simulink library "casper_library_misc"  (Simulink 8.0)
settings: Solver=ode45  SolverMode=SingleTasking  StartTime=0.0  StopTime=10.0  RelTol=1e-3
libraries: xbsIndex_r4 x255, casper_library_misc x8, xps_library x6, simulink x4
(part 3 of 3)

== system casper_library_misc/complex_convert/ri_to_c ==
  re : Inport
  im : Inport  Port=2
  concat : xbsIndex_r4/Concat  num_inputs=2  dbl_ovrd=off  block_type=concat
      settings: block_version=9.1.01
  force_im : xbsIndex_r4/Reinterpret  force_arith_type=on  arith_type=Unsigned  force_bin_pt=on  bin_pt=0  block_type=reinterpret
      settings: infoedit="Changes signal type without altering the binary representation.   You can changed the signal between signed and unsigned, and relocate the binary point.<P><P>Hardware notes: In hardware this block costs nothing.<P><P>Example:  Suppose the input is 6 bits wide, signed, with 2 fractional bits, and the output is forced to unsigned with 0 fractional bits.  Then an input of -2.0 (1110.00 in binary 2's complement) becomes an output of 56 (111000 in binary)."  block_version=9.1.01
  force_re : xbsIndex_r4/Reinterpret  force_arith_type=on  arith_type=Unsigned  force_bin_pt=on  bin_pt=0  block_type=reinterpret
      settings: infoedit="Changes signal type without altering the binary representation.   You can changed the signal between signed and unsigned, and relocate the binary point.<P><P>Hardware notes: In hardware this block costs nothing.<P><P>Example:  Suppose the input is 6 bits wide, signed, with 2 fractional bits, and the output is forced to unsigned with 0 fractional bits.  Then an input of -2.0 (1110.00 in binary 2's complement) becomes an output of 56 (111000 in binary)."  block_version=9.1.01
  c : Outport
  wires:
  force_re/1 -> concat/1
  force_im/1 -> concat/2
  re/1 -> force_re/1
  concat/1 -> c/1
  im/1 -> force_im/1

== system casper_library_misc/pulse_ext/posedge ==
  In : Inport
  Delay : xbsIndex_r4/Delay  rst=off  infoeditControl=Selection of Reset will increase slice count due to use of real FFs and instead of SRLs  en=off  latency=1  dbl_ovrd=off  reg_retiming=on  block_type=delay
      settings: xl_area=[0, 0, 0, 0, 0, 0, 0]  block_version=9.1.01
  Inverter : xbsIndex_r4/Inverter  en=off  latency=0  dbl_ovrd=off  block_type=inv
      settings: xl_area=[0, 0, 0, 0, 0, 0, 0]  block_version=9.1.01
  Logical : xbsIndex_r4/Logical  logical_function=AND  inputs=2  en=off  latency=0  precision=Full  arith_type=Unsigned  n_bits=8  bin_pt=2  align_bp=on  dbl_ovrd=off  block_type=logical
      settings: xl_area=[0, 0, 0, 0, 0, 0, 0]  block_version=9.1.01
  Out : Outport
  wires:
  Logical/1 -> Out/1
  In/1 -> Logical/2, Delay/1
  Inverter/1 -> Logical/1
  Delay/1 -> Inverter/1

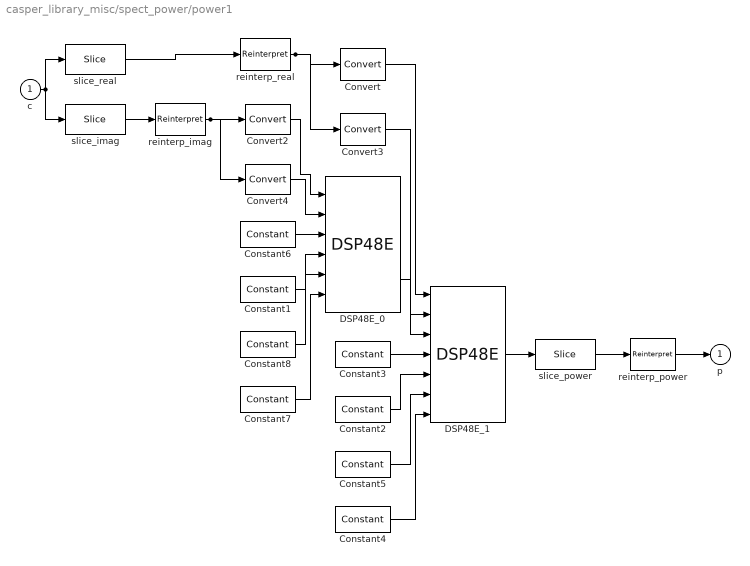
== system casper_library_misc/spect_power/power1 ==
  c : Inport
  Constant1 : xbsIndex_r4/Constant  const=0  gui_display_data_type=Fixed-point  arith_type=Unsigned  n_bits=4  bin_pt=0  preci_type=Single  exp_width=8  frac_width=24  explicit_period=off  period=1  equ=P=C  opselect=C  inp2=PCIN>>17  opr=+  inp1=P  carry=CIN  dbl_ovrd=off  block_type=constant
      settings: block_version=11.4
  Constant2 : xbsIndex_r4/Constant  const=0  gui_display_data_type=Fixed-point  arith_type=Unsigned  n_bits=4  bin_pt=0  preci_type=Single  exp_width=8  frac_width=24  explicit_period=off  period=1  equ=P=C  opselect=C  inp2=PCIN>>17  opr=+  inp1=P  carry=CIN  dbl_ovrd=off  block_type=constant
      settings: block_version=11.4
  Constant3 : xbsIndex_r4/Constant  const=21  gui_display_data_type=Fixed-point  arith_type=Unsigned  n_bits=7  bin_pt=0  preci_type=Single  exp_width=8  frac_width=24  explicit_period=off  period=1  equ=P=C  opselect=C  inp2=PCIN>>17  opr=+  inp1=P  carry=CIN  dbl_ovrd=off  block_type=constant
      settings: block_version=11.4
  Constant4 : xbsIndex_r4/Constant  const=0  gui_display_data_type=Fixed-point  arith_type=Unsigned  n_bits=3  bin_pt=0  preci_type=Single  exp_width=8  frac_width=24  explicit_period=off  period=1  equ=P=C  opselect=C  inp2=PCIN>>17  opr=+  inp1=P  carry=CIN  dbl_ovrd=off  block_type=constant
      settings: block_version=11.4
  Constant5 : xbsIndex_r4/Constant  const=0  gui_display_data_type=Fixed-point  arith_type=Unsigned  n_bits=1  bin_pt=0  preci_type=Single  exp_width=8  frac_width=24  explicit_period=off  period=1  equ=P=C  opselect=C  inp2=PCIN>>17  opr=+  inp1=P  carry=CIN  dbl_ovrd=off  block_type=constant
      settings: block_version=11.4
  Constant6 : xbsIndex_r4/Constant  const=5  gui_display_data_type=Fixed-point  arith_type=Unsigned  n_bits=7  bin_pt=0  preci_type=Single  exp_width=8  frac_width=24  explicit_period=off  period=1  equ=P=C  opselect=C  inp2=PCIN>>17  opr=+  inp1=P  carry=CIN  dbl_ovrd=off  block_type=constant
      settings: block_version=11.4
  Constant7 : xbsIndex_r4/Constant  const=0  gui_display_data_type=Fixed-point  arith_type=Unsigned  n_bits=3  bin_pt=0  preci_type=Single  exp_width=8  frac_width=24  explicit_period=off  period=1  equ=P=C  opselect=C  inp2=PCIN>>17  opr=+  inp1=P  carry=CIN  dbl_ovrd=off  block_type=constant
      settings: block_version=11.4
  Constant8 : xbsIndex_r4/Constant  const=0  gui_display_data_type=Fixed-point  arith_type=Unsigned  n_bits=1  bin_pt=0  preci_type=Single  exp_width=8  frac_width=24  explicit_period=off  period=1  equ=P=C  opselect=C  inp2=PCIN>>17  opr=+  inp1=P  carry=CIN  dbl_ovrd=off  block_type=constant
      settings: block_version=11.4
  Convert : xbsIndex_r4/Convert  gui_display_data_type=Fixed-point  arith_type="Signed  (2's comp)"  n_bits=30  bin_pt=0  float_type=Single  exp_bits=8  fraction_bits=24  quantization=Truncate  overflow=Wrap  en=off  latency=0  dbl_ovrd=off  pipeline=off  block_type=convert
      settings: block_version=11.4
  Convert2 : xbsIndex_r4/Convert  gui_display_data_type=Fixed-point  arith_type="Signed  (2's comp)"  n_bits=30  bin_pt=0  float_type=Single  exp_bits=8  fraction_bits=24  quantization=Truncate  overflow=Wrap  en=off  latency=0  dbl_ovrd=off  pipeline=off  block_type=convert
      settings: block_version=11.4
  Convert3 : xbsIndex_r4/Convert  gui_display_data_type=Fixed-point  arith_type="Signed  (2's comp)"  n_bits=18  bin_pt=0  float_type=Single  exp_bits=8  fraction_bits=24  quantization=Truncate  overflow=Wrap  en=off  latency=0  dbl_ovrd=off  pipeline=off  block_type=convert
      settings: block_version=11.4
  Convert4 : xbsIndex_r4/Convert  gui_display_data_type=Fixed-point  arith_type="Signed  (2's comp)"  n_bits=18  bin_pt=0  float_type=Single  exp_bits=8  fraction_bits=24  quantization=Truncate  overflow=Wrap  en=off  latency=0  dbl_ovrd=off  pipeline=off  block_type=convert
      settings: block_version=11.4
  DSP48E_0 : xbsIndex_r4/DSP48E  use_a=Direct from A Port  use_b=Direct from B Port  reset_preg=off  pattern_from_creg=off  pattern='000000000000'  mask_from_creg=off  pattern_mask='3FFFFFFFFFFF'  sel_rounding_mask=Select mask  use_op=off  use_creg=off  rst_all=off  en_all=off  use_pcin=off  use_carrycascin=off  use_multsignin=off  use_carryout=off  use_patterndetect=off  use_patternbdetect=off  use_overflow=off  use_underflow=off  use_acout=off  use_bcout=off  use_pcout=on  use_multsignout=off  use_carrycascout=off  pipeline_a=1  pipeline_b=1  pipeline_acout=1  pipeline_bcout=1  pipeline_c=on  pipeline_p=on  pipeline_mult=on  pipeline_opmode=on  pipeline_alumode=on  pipeline_carryin=on  pipeline_carryinsel=on  rst_a=off  rst_b=off  rst_c=off  rst_mult=off  rst_p=off  rst_carry_in=off  rst_alumode=off  rst_ctrl=off  en_a1=off  en_a2=off  en_b1=off  en_b2=off  en_c=off  en_mult=off  en_p=off  en_carry_in=off  en_alumode=off  en_multcarryin=off  en_ctrl=off  use_synth_model=off  addsub_mode=ONE48  xl_useadderonly=off  block_type=dsp48e
      settings: block_version=11.4
  DSP48E_1 : xbsIndex_r4/DSP48E  use_a=Direct from A Port  use_b=Direct from B Port  reset_preg=off  pattern_from_creg=off  pattern='000000000000'  mask_from_creg=off  pattern_mask='3FFFFFFFFFFF'  sel_rounding_mask=Select mask  use_op=off  use_creg=off  rst_all=off  en_all=off  use_pcin=on  use_carrycascin=off  use_multsignin=off  use_carryout=off  use_patterndetect=off  use_patternbdetect=off  use_overflow=off  use_underflow=off  use_acout=off  use_bcout=off  use_pcout=off  use_multsignout=off  use_carrycascout=off  pipeline_a=2  pipeline_b=2  pipeline_acout=1  pipeline_bcout=1  pipeline_c=on  pipeline_p=on  pipeline_mult=on  pipeline_opmode=on  pipeline_alumode=on  pipeline_carryin=on  pipeline_carryinsel=on  rst_a=off  rst_b=off  rst_c=off  rst_mult=off  rst_p=off  rst_carry_in=off  rst_alumode=off  rst_ctrl=off  en_a1=off  en_a2=off  en_b1=off  en_b2=off  en_c=off  en_mult=off  en_p=off  en_carry_in=off  en_alumode=off  en_multcarryin=off  en_ctrl=off  use_synth_model=off  addsub_mode=ONE48  xl_useadderonly=off  block_type=dsp48e
      settings: block_version=11.4
  reinterp_imag : xbsIndex_r4/Reinterpret  force_arith_type=on  arith_type="Signed  (2's comp)"  force_bin_pt=off  bin_pt=0  block_type=reinterpret
      settings: infoedit="Changes signal type without altering the binary representation.   You can changed the signal between signed and unsigned, and relocate the binary point.<br><br>Hardware notes: In hardware this block costs nothing.<br><br>Example:  Suppose the input is 6 bits wide, signed, with 2 fractional bits, and the output is forced to unsigned with 0 fractional bits.  Then an input of -2.0 (1110.00 in binary 2's complement) becomes an output of 56 (111000 in binary)."
  reinterp_power : xbsIndex_r4/Reinterpret  force_arith_type=on  arith_type=Unsigned  force_bin_pt=on  bin_pt=34  block_type=reinterpret
      settings: infoedit="Changes signal type without altering the binary representation.   You can changed the signal between signed and unsigned, and relocate the binary point.<br><br>Hardware notes: In hardware this block costs nothing.<br><br>Example:  Suppose the input is 6 bits wide, signed, with 2 fractional bits, and the output is forced to unsigned with 0 fractional bits.  Then an input of -2.0 (1110.00 in binary 2's complement) becomes an output of 56 (111000 in binary)."
  reinterp_real : xbsIndex_r4/Reinterpret  force_arith_type=on  arith_type="Signed  (2's comp)"  force_bin_pt=off  bin_pt=0  block_type=reinterpret
      settings: infoedit="Changes signal type without altering the binary representation.   You can changed the signal between signed and unsigned, and relocate the binary point.<br><br>Hardware notes: In hardware this block costs nothing.<br><br>Example:  Suppose the input is 6 bits wide, signed, with 2 fractional bits, and the output is forced to unsigned with 0 fractional bits.  Then an input of -2.0 (1110.00 in binary 2's complement) becomes an output of 56 (111000 in binary)."
  slice_imag : xbsIndex_r4/Slice  nbits=18  boolean_output=off  mode=Lower Bit Location + Width  bit1=0  base1=MSB of Input  bit0=0  base0=LSB of Input  dbl_ovrd=off  block_type=slice
  slice_power : xbsIndex_r4/Slice  nbits=36  boolean_output=off  mode=Lower Bit Location + Width  bit1=0  base1=MSB of Input  bit0=0  base0=LSB of Input  dbl_ovrd=off  block_type=slice
  slice_real : xbsIndex_r4/Slice  nbits=18  boolean_output=off  mode=Upper Bit Location + Width  bit1=0  base1=MSB of Input  bit0=0  base0=LSB of Input  dbl_ovrd=off  block_type=slice
  p : Outport
  wires:
  reinterp_imag/1 -> Convert4/1, Convert2/1
  reinterp_real/1 -> Convert3/1, Convert/1
  c/1 -> slice_real/1, slice_imag/1
  slice_real/1 -> reinterp_real/1
  slice_power/1 -> reinterp_power/1
  DSP48E_1/1 -> slice_power/1
  slice_imag/1 -> reinterp_imag/1
  reinterp_power/1 -> p/1
  Constant4/1 -> DSP48E_1/7
  Constant5/1 -> DSP48E_1/6
  Constant2/1 -> DSP48E_1/5
  Constant3/1 -> DSP48E_1/4
  DSP48E_0/2 -> DSP48E_1/3
  Convert3/1 -> DSP48E_1/2
  Convert/1 -> DSP48E_1/1
  Constant7/1 -> DSP48E_0/6
  Constant8/1 -> DSP48E_0/5
  Constant1/1 -> DSP48E_0/4
  Constant6/1 -> DSP48E_0/3
  Convert4/1 -> DSP48E_0/2
  Convert2/1 -> DSP48E_0/1

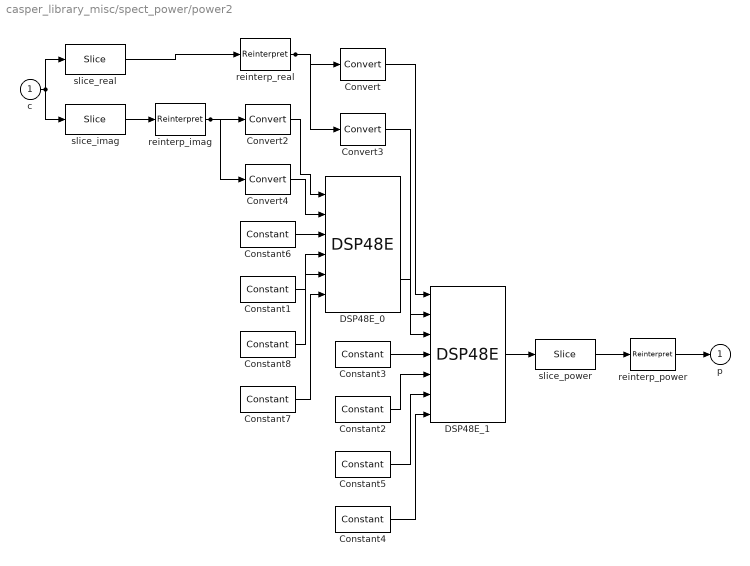
== system casper_library_misc/spect_power/power2 ==
  c : Inport
  Constant1 : xbsIndex_r4/Constant  const=0  gui_display_data_type=Fixed-point  arith_type=Unsigned  n_bits=4  bin_pt=0  preci_type=Single  exp_width=8  frac_width=24  explicit_period=off  period=1  equ=P=C  opselect=C  inp2=PCIN>>17  opr=+  inp1=P  carry=CIN  dbl_ovrd=off  block_type=constant
      settings: block_version=11.4
  Constant2 : xbsIndex_r4/Constant  const=0  gui_display_data_type=Fixed-point  arith_type=Unsigned  n_bits=4  bin_pt=0  preci_type=Single  exp_width=8  frac_width=24  explicit_period=off  period=1  equ=P=C  opselect=C  inp2=PCIN>>17  opr=+  inp1=P  carry=CIN  dbl_ovrd=off  block_type=constant
      settings: block_version=11.4
  Constant3 : xbsIndex_r4/Constant  const=21  gui_display_data_type=Fixed-point  arith_type=Unsigned  n_bits=7  bin_pt=0  preci_type=Single  exp_width=8  frac_width=24  explicit_period=off  period=1  equ=P=C  opselect=C  inp2=PCIN>>17  opr=+  inp1=P  carry=CIN  dbl_ovrd=off  block_type=constant
      settings: block_version=11.4
  Constant4 : xbsIndex_r4/Constant  const=0  gui_display_data_type=Fixed-point  arith_type=Unsigned  n_bits=3  bin_pt=0  preci_type=Single  exp_width=8  frac_width=24  explicit_period=off  period=1  equ=P=C  opselect=C  inp2=PCIN>>17  opr=+  inp1=P  carry=CIN  dbl_ovrd=off  block_type=constant
      settings: block_version=11.4
  Constant5 : xbsIndex_r4/Constant  const=0  gui_display_data_type=Fixed-point  arith_type=Unsigned  n_bits=1  bin_pt=0  preci_type=Single  exp_width=8  frac_width=24  explicit_period=off  period=1  equ=P=C  opselect=C  inp2=PCIN>>17  opr=+  inp1=P  carry=CIN  dbl_ovrd=off  block_type=constant
      settings: block_version=11.4
  Constant6 : xbsIndex_r4/Constant  const=5  gui_display_data_type=Fixed-point  arith_type=Unsigned  n_bits=7  bin_pt=0  preci_type=Single  exp_width=8  frac_width=24  explicit_period=off  period=1  equ=P=C  opselect=C  inp2=PCIN>>17  opr=+  inp1=P  carry=CIN  dbl_ovrd=off  block_type=constant
      settings: block_version=11.4
  Constant7 : xbsIndex_r4/Constant  const=0  gui_display_data_type=Fixed-point  arith_type=Unsigned  n_bits=3  bin_pt=0  preci_type=Single  exp_width=8  frac_width=24  explicit_period=off  period=1  equ=P=C  opselect=C  inp2=PCIN>>17  opr=+  inp1=P  carry=CIN  dbl_ovrd=off  block_type=constant
      settings: block_version=11.4
  Constant8 : xbsIndex_r4/Constant  const=0  gui_display_data_type=Fixed-point  arith_type=Unsigned  n_bits=1  bin_pt=0  preci_type=Single  exp_width=8  frac_width=24  explicit_period=off  period=1  equ=P=C  opselect=C  inp2=PCIN>>17  opr=+  inp1=P  carry=CIN  dbl_ovrd=off  block_type=constant
      settings: block_version=11.4
  Convert : xbsIndex_r4/Convert  gui_display_data_type=Fixed-point  arith_type="Signed  (2's comp)"  n_bits=30  bin_pt=0  float_type=Single  exp_bits=8  fraction_bits=24  quantization=Truncate  overflow=Wrap  en=off  latency=0  dbl_ovrd=off  pipeline=off  block_type=convert
      settings: block_version=11.4
  Convert2 : xbsIndex_r4/Convert  gui_display_data_type=Fixed-point  arith_type="Signed  (2's comp)"  n_bits=30  bin_pt=0  float_type=Single  exp_bits=8  fraction_bits=24  quantization=Truncate  overflow=Wrap  en=off  latency=0  dbl_ovrd=off  pipeline=off  block_type=convert
      settings: block_version=11.4
  Convert3 : xbsIndex_r4/Convert  gui_display_data_type=Fixed-point  arith_type="Signed  (2's comp)"  n_bits=18  bin_pt=0  float_type=Single  exp_bits=8  fraction_bits=24  quantization=Truncate  overflow=Wrap  en=off  latency=0  dbl_ovrd=off  pipeline=off  block_type=convert
      settings: block_version=11.4
  Convert4 : xbsIndex_r4/Convert  gui_display_data_type=Fixed-point  arith_type="Signed  (2's comp)"  n_bits=18  bin_pt=0  float_type=Single  exp_bits=8  fraction_bits=24  quantization=Truncate  overflow=Wrap  en=off  latency=0  dbl_ovrd=off  pipeline=off  block_type=convert
      settings: block_version=11.4
  DSP48E_0 : xbsIndex_r4/DSP48E  use_a=Direct from A Port  use_b=Direct from B Port  reset_preg=off  pattern_from_creg=off  pattern='000000000000'  mask_from_creg=off  pattern_mask='3FFFFFFFFFFF'  sel_rounding_mask=Select mask  use_op=off  use_creg=off  rst_all=off  en_all=off  use_pcin=off  use_carrycascin=off  use_multsignin=off  use_carryout=off  use_patterndetect=off  use_patternbdetect=off  use_overflow=off  use_underflow=off  use_acout=off  use_bcout=off  use_pcout=on  use_multsignout=off  use_carrycascout=off  pipeline_a=1  pipeline_b=1  pipeline_acout=1  pipeline_bcout=1  pipeline_c=on  pipeline_p=on  pipeline_mult=on  pipeline_opmode=on  pipeline_alumode=on  pipeline_carryin=on  pipeline_carryinsel=on  rst_a=off  rst_b=off  rst_c=off  rst_mult=off  rst_p=off  rst_carry_in=off  rst_alumode=off  rst_ctrl=off  en_a1=off  en_a2=off  en_b1=off  en_b2=off  en_c=off  en_mult=off  en_p=off  en_carry_in=off  en_alumode=off  en_multcarryin=off  en_ctrl=off  use_synth_model=off  addsub_mode=ONE48  xl_useadderonly=off  block_type=dsp48e
      settings: block_version=11.4
  DSP48E_1 : xbsIndex_r4/DSP48E  use_a=Direct from A Port  use_b=Direct from B Port  reset_preg=off  pattern_from_creg=off  pattern='000000000000'  mask_from_creg=off  pattern_mask='3FFFFFFFFFFF'  sel_rounding_mask=Select mask  use_op=off  use_creg=off  rst_all=off  en_all=off  use_pcin=on  use_carrycascin=off  use_multsignin=off  use_carryout=off  use_patterndetect=off  use_patternbdetect=off  use_overflow=off  use_underflow=off  use_acout=off  use_bcout=off  use_pcout=off  use_multsignout=off  use_carrycascout=off  pipeline_a=2  pipeline_b=2  pipeline_acout=1  pipeline_bcout=1  pipeline_c=on  pipeline_p=on  pipeline_mult=on  pipeline_opmode=on  pipeline_alumode=on  pipeline_carryin=on  pipeline_carryinsel=on  rst_a=off  rst_b=off  rst_c=off  rst_mult=off  rst_p=off  rst_carry_in=off  rst_alumode=off  rst_ctrl=off  en_a1=off  en_a2=off  en_b1=off  en_b2=off  en_c=off  en_mult=off  en_p=off  en_carry_in=off  en_alumode=off  en_multcarryin=off  en_ctrl=off  use_synth_model=off  addsub_mode=ONE48  xl_useadderonly=off  block_type=dsp48e
      settings: block_version=11.4
  reinterp_imag : xbsIndex_r4/Reinterpret  force_arith_type=on  arith_type="Signed  (2's comp)"  force_bin_pt=off  bin_pt=0  block_type=reinterpret
      settings: infoedit="Changes signal type without altering the binary representation.   You can changed the signal between signed and unsigned, and relocate the binary point.<br><br>Hardware notes: In hardware this block costs nothing.<br><br>Example:  Suppose the input is 6 bits wide, signed, with 2 fractional bits, and the output is forced to unsigned with 0 fractional bits.  Then an input of -2.0 (1110.00 in binary 2's complement) becomes an output of 56 (111000 in binary)."
  reinterp_power : xbsIndex_r4/Reinterpret  force_arith_type=on  arith_type=Unsigned  force_bin_pt=on  bin_pt=34  block_type=reinterpret
      settings: infoedit="Changes signal type without altering the binary representation.   You can changed the signal between signed and unsigned, and relocate the binary point.<br><br>Hardware notes: In hardware this block costs nothing.<br><br>Example:  Suppose the input is 6 bits wide, signed, with 2 fractional bits, and the output is forced to unsigned with 0 fractional bits.  Then an input of -2.0 (1110.00 in binary 2's complement) becomes an output of 56 (111000 in binary)."
  reinterp_real : xbsIndex_r4/Reinterpret  force_arith_type=on  arith_type="Signed  (2's comp)"  force_bin_pt=off  bin_pt=0  block_type=reinterpret
      settings: infoedit="Changes signal type without altering the binary representation.   You can changed the signal between signed and unsigned, and relocate the binary point.<br><br>Hardware notes: In hardware this block costs nothing.<br><br>Example:  Suppose the input is 6 bits wide, signed, with 2 fractional bits, and the output is forced to unsigned with 0 fractional bits.  Then an input of -2.0 (1110.00 in binary 2's complement) becomes an output of 56 (111000 in binary)."
  slice_imag : xbsIndex_r4/Slice  nbits=18  boolean_output=off  mode=Lower Bit Location + Width  bit1=0  base1=MSB of Input  bit0=0  base0=LSB of Input  dbl_ovrd=off  block_type=slice
  slice_power : xbsIndex_r4/Slice  nbits=36  boolean_output=off  mode=Lower Bit Location + Width  bit1=0  base1=MSB of Input  bit0=0  base0=LSB of Input  dbl_ovrd=off  block_type=slice
  slice_real : xbsIndex_r4/Slice  nbits=18  boolean_output=off  mode=Upper Bit Location + Width  bit1=0  base1=MSB of Input  bit0=0  base0=LSB of Input  dbl_ovrd=off  block_type=slice
  p : Outport
  wires:
  reinterp_imag/1 -> Convert4/1, Convert2/1
  reinterp_real/1 -> Convert3/1, Convert/1
  c/1 -> slice_real/1, slice_imag/1
  slice_real/1 -> reinterp_real/1
  slice_power/1 -> reinterp_power/1
  DSP48E_1/1 -> slice_power/1
  slice_imag/1 -> reinterp_imag/1
  reinterp_power/1 -> p/1
  Constant4/1 -> DSP48E_1/7
  Constant5/1 -> DSP48E_1/6
  Constant2/1 -> DSP48E_1/5
  Constant3/1 -> DSP48E_1/4
  DSP48E_0/2 -> DSP48E_1/3
  Convert3/1 -> DSP48E_1/2
  Convert/1 -> DSP48E_1/1
  Constant7/1 -> DSP48E_0/6
  Constant8/1 -> DSP48E_0/5
  Constant1/1 -> DSP48E_0/4
  Constant6/1 -> DSP48E_0/3
  Convert4/1 -> DSP48E_0/2
  Convert2/1 -> DSP48E_0/1

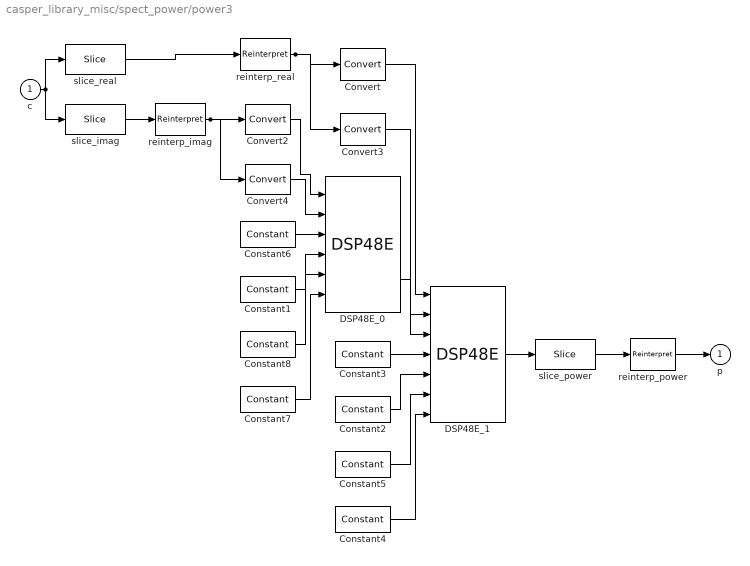
== system casper_library_misc/spect_power/power3 ==
  c : Inport
  Constant1 : xbsIndex_r4/Constant  const=0  gui_display_data_type=Fixed-point  arith_type=Unsigned  n_bits=4  bin_pt=0  preci_type=Single  exp_width=8  frac_width=24  explicit_period=off  period=1  equ=P=C  opselect=C  inp2=PCIN>>17  opr=+  inp1=P  carry=CIN  dbl_ovrd=off  block_type=constant
      settings: block_version=11.4
  Constant2 : xbsIndex_r4/Constant  const=0  gui_display_data_type=Fixed-point  arith_type=Unsigned  n_bits=4  bin_pt=0  preci_type=Single  exp_width=8  frac_width=24  explicit_period=off  period=1  equ=P=C  opselect=C  inp2=PCIN>>17  opr=+  inp1=P  carry=CIN  dbl_ovrd=off  block_type=constant
      settings: block_version=11.4
  Constant3 : xbsIndex_r4/Constant  const=21  gui_display_data_type=Fixed-point  arith_type=Unsigned  n_bits=7  bin_pt=0  preci_type=Single  exp_width=8  frac_width=24  explicit_period=off  period=1  equ=P=C  opselect=C  inp2=PCIN>>17  opr=+  inp1=P  carry=CIN  dbl_ovrd=off  block_type=constant
      settings: block_version=11.4
  Constant4 : xbsIndex_r4/Constant  const=0  gui_display_data_type=Fixed-point  arith_type=Unsigned  n_bits=3  bin_pt=0  preci_type=Single  exp_width=8  frac_width=24  explicit_period=off  period=1  equ=P=C  opselect=C  inp2=PCIN>>17  opr=+  inp1=P  carry=CIN  dbl_ovrd=off  block_type=constant
      settings: block_version=11.4
  Constant5 : xbsIndex_r4/Constant  const=0  gui_display_data_type=Fixed-point  arith_type=Unsigned  n_bits=1  bin_pt=0  preci_type=Single  exp_width=8  frac_width=24  explicit_period=off  period=1  equ=P=C  opselect=C  inp2=PCIN>>17  opr=+  inp1=P  carry=CIN  dbl_ovrd=off  block_type=constant
      settings: block_version=11.4
  Constant6 : xbsIndex_r4/Constant  const=5  gui_display_data_type=Fixed-point  arith_type=Unsigned  n_bits=7  bin_pt=0  preci_type=Single  exp_width=8  frac_width=24  explicit_period=off  period=1  equ=P=C  opselect=C  inp2=PCIN>>17  opr=+  inp1=P  carry=CIN  dbl_ovrd=off  block_type=constant
      settings: block_version=11.4
  Constant7 : xbsIndex_r4/Constant  const=0  gui_display_data_type=Fixed-point  arith_type=Unsigned  n_bits=3  bin_pt=0  preci_type=Single  exp_width=8  frac_width=24  explicit_period=off  period=1  equ=P=C  opselect=C  inp2=PCIN>>17  opr=+  inp1=P  carry=CIN  dbl_ovrd=off  block_type=constant
      settings: block_version=11.4
  Constant8 : xbsIndex_r4/Constant  const=0  gui_display_data_type=Fixed-point  arith_type=Unsigned  n_bits=1  bin_pt=0  preci_type=Single  exp_width=8  frac_width=24  explicit_period=off  period=1  equ=P=C  opselect=C  inp2=PCIN>>17  opr=+  inp1=P  carry=CIN  dbl_ovrd=off  block_type=constant
      settings: block_version=11.4
  Convert : xbsIndex_r4/Convert  gui_display_data_type=Fixed-point  arith_type="Signed  (2's comp)"  n_bits=30  bin_pt=0  float_type=Single  exp_bits=8  fraction_bits=24  quantization=Truncate  overflow=Wrap  en=off  latency=0  dbl_ovrd=off  pipeline=off  block_type=convert
      settings: block_version=11.4
  Convert2 : xbsIndex_r4/Convert  gui_display_data_type=Fixed-point  arith_type="Signed  (2's comp)"  n_bits=30  bin_pt=0  float_type=Single  exp_bits=8  fraction_bits=24  quantization=Truncate  overflow=Wrap  en=off  latency=0  dbl_ovrd=off  pipeline=off  block_type=convert
      settings: block_version=11.4
  Convert3 : xbsIndex_r4/Convert  gui_display_data_type=Fixed-point  arith_type="Signed  (2's comp)"  n_bits=18  bin_pt=0  float_type=Single  exp_bits=8  fraction_bits=24  quantization=Truncate  overflow=Wrap  en=off  latency=0  dbl_ovrd=off  pipeline=off  block_type=convert
      settings: block_version=11.4
  Convert4 : xbsIndex_r4/Convert  gui_display_data_type=Fixed-point  arith_type="Signed  (2's comp)"  n_bits=18  bin_pt=0  float_type=Single  exp_bits=8  fraction_bits=24  quantization=Truncate  overflow=Wrap  en=off  latency=0  dbl_ovrd=off  pipeline=off  block_type=convert
      settings: block_version=11.4
  DSP48E_0 : xbsIndex_r4/DSP48E  use_a=Direct from A Port  use_b=Direct from B Port  reset_preg=off  pattern_from_creg=off  pattern='000000000000'  mask_from_creg=off  pattern_mask='3FFFFFFFFFFF'  sel_rounding_mask=Select mask  use_op=off  use_creg=off  rst_all=off  en_all=off  use_pcin=off  use_carrycascin=off  use_multsignin=off  use_carryout=off  use_patterndetect=off  use_patternbdetect=off  use_overflow=off  use_underflow=off  use_acout=off  use_bcout=off  use_pcout=on  use_multsignout=off  use_carrycascout=off  pipeline_a=1  pipeline_b=1  pipeline_acout=1  pipeline_bcout=1  pipeline_c=on  pipeline_p=on  pipeline_mult=on  pipeline_opmode=on  pipeline_alumode=on  pipeline_carryin=on  pipeline_carryinsel=on  rst_a=off  rst_b=off  rst_c=off  rst_mult=off  rst_p=off  rst_carry_in=off  rst_alumode=off  rst_ctrl=off  en_a1=off  en_a2=off  en_b1=off  en_b2=off  en_c=off  en_mult=off  en_p=off  en_carry_in=off  en_alumode=off  en_multcarryin=off  en_ctrl=off  use_synth_model=off  addsub_mode=ONE48  xl_useadderonly=off  block_type=dsp48e
      settings: block_version=11.4
  DSP48E_1 : xbsIndex_r4/DSP48E  use_a=Direct from A Port  use_b=Direct from B Port  reset_preg=off  pattern_from_creg=off  pattern='000000000000'  mask_from_creg=off  pattern_mask='3FFFFFFFFFFF'  sel_rounding_mask=Select mask  use_op=off  use_creg=off  rst_all=off  en_all=off  use_pcin=on  use_carrycascin=off  use_multsignin=off  use_carryout=off  use_patterndetect=off  use_patternbdetect=off  use_overflow=off  use_underflow=off  use_acout=off  use_bcout=off  use_pcout=off  use_multsignout=off  use_carrycascout=off  pipeline_a=2  pipeline_b=2  pipeline_acout=1  pipeline_bcout=1  pipeline_c=on  pipeline_p=on  pipeline_mult=on  pipeline_opmode=on  pipeline_alumode=on  pipeline_carryin=on  pipeline_carryinsel=on  rst_a=off  rst_b=off  rst_c=off  rst_mult=off  rst_p=off  rst_carry_in=off  rst_alumode=off  rst_ctrl=off  en_a1=off  en_a2=off  en_b1=off  en_b2=off  en_c=off  en_mult=off  en_p=off  en_carry_in=off  en_alumode=off  en_multcarryin=off  en_ctrl=off  use_synth_model=off  addsub_mode=ONE48  xl_useadderonly=off  block_type=dsp48e
      settings: block_version=11.4
  reinterp_imag : xbsIndex_r4/Reinterpret  force_arith_type=on  arith_type="Signed  (2's comp)"  force_bin_pt=off  bin_pt=0  block_type=reinterpret
      settings: infoedit="Changes signal type without altering the binary representation.   You can changed the signal between signed and unsigned, and relocate the binary point.<br><br>Hardware notes: In hardware this block costs nothing.<br><br>Example:  Suppose the input is 6 bits wide, signed, with 2 fractional bits, and the output is forced to unsigned with 0 fractional bits.  Then an input of -2.0 (1110.00 in binary 2's complement) becomes an output of 56 (111000 in binary)."
  reinterp_power : xbsIndex_r4/Reinterpret  force_arith_type=on  arith_type=Unsigned  force_bin_pt=on  bin_pt=34  block_type=reinterpret
      settings: infoedit="Changes signal type without altering the binary representation.   You can changed the signal between signed and unsigned, and relocate the binary point.<br><br>Hardware notes: In hardware this block costs nothing.<br><br>Example:  Suppose the input is 6 bits wide, signed, with 2 fractional bits, and the output is forced to unsigned with 0 fractional bits.  Then an input of -2.0 (1110.00 in binary 2's complement) becomes an output of 56 (111000 in binary)."
  reinterp_real : xbsIndex_r4/Reinterpret  force_arith_type=on  arith_type="Signed  (2's comp)"  force_bin_pt=off  bin_pt=0  block_type=reinterpret
      settings: infoedit="Changes signal type without altering the binary representation.   You can changed the signal between signed and unsigned, and relocate the binary point.<br><br>Hardware notes: In hardware this block costs nothing.<br><br>Example:  Suppose the input is 6 bits wide, signed, with 2 fractional bits, and the output is forced to unsigned with 0 fractional bits.  Then an input of -2.0 (1110.00 in binary 2's complement) becomes an output of 56 (111000 in binary)."
  slice_imag : xbsIndex_r4/Slice  nbits=18  boolean_output=off  mode=Lower Bit Location + Width  bit1=0  base1=MSB of Input  bit0=0  base0=LSB of Input  dbl_ovrd=off  block_type=slice
  slice_power : xbsIndex_r4/Slice  nbits=36  boolean_output=off  mode=Lower Bit Location + Width  bit1=0  base1=MSB of Input  bit0=0  base0=LSB of Input  dbl_ovrd=off  block_type=slice
  slice_real : xbsIndex_r4/Slice  nbits=18  boolean_output=off  mode=Upper Bit Location + Width  bit1=0  base1=MSB of Input  bit0=0  base0=LSB of Input  dbl_ovrd=off  block_type=slice
  p : Outport
  wires:
  reinterp_imag/1 -> Convert4/1, Convert2/1
  reinterp_real/1 -> Convert3/1, Convert/1
  c/1 -> slice_real/1, slice_imag/1
  slice_real/1 -> reinterp_real/1
  slice_power/1 -> reinterp_power/1
  DSP48E_1/1 -> slice_power/1
  slice_imag/1 -> reinterp_imag/1
  reinterp_power/1 -> p/1
  Constant4/1 -> DSP48E_1/7
  Constant5/1 -> DSP48E_1/6
  Constant2/1 -> DSP48E_1/5
  Constant3/1 -> DSP48E_1/4
  DSP48E_0/2 -> DSP48E_1/3
  Convert3/1 -> DSP48E_1/2
  Convert/1 -> DSP48E_1/1
  Constant7/1 -> DSP48E_0/6
  Constant8/1 -> DSP48E_0/5
  Constant1/1 -> DSP48E_0/4
  Constant6/1 -> DSP48E_0/3
  Convert4/1 -> DSP48E_0/2
  Convert2/1 -> DSP48E_0/1

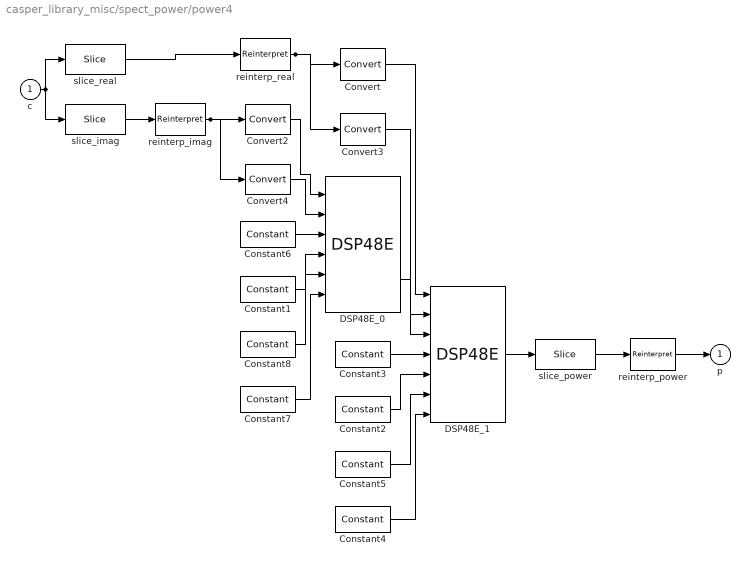
== system casper_library_misc/spect_power/power4 ==
  c : Inport
  Constant1 : xbsIndex_r4/Constant  const=0  gui_display_data_type=Fixed-point  arith_type=Unsigned  n_bits=4  bin_pt=0  preci_type=Single  exp_width=8  frac_width=24  explicit_period=off  period=1  equ=P=C  opselect=C  inp2=PCIN>>17  opr=+  inp1=P  carry=CIN  dbl_ovrd=off  block_type=constant
      settings: block_version=11.4
  Constant2 : xbsIndex_r4/Constant  const=0  gui_display_data_type=Fixed-point  arith_type=Unsigned  n_bits=4  bin_pt=0  preci_type=Single  exp_width=8  frac_width=24  explicit_period=off  period=1  equ=P=C  opselect=C  inp2=PCIN>>17  opr=+  inp1=P  carry=CIN  dbl_ovrd=off  block_type=constant
      settings: block_version=11.4
  Constant3 : xbsIndex_r4/Constant  const=21  gui_display_data_type=Fixed-point  arith_type=Unsigned  n_bits=7  bin_pt=0  preci_type=Single  exp_width=8  frac_width=24  explicit_period=off  period=1  equ=P=C  opselect=C  inp2=PCIN>>17  opr=+  inp1=P  carry=CIN  dbl_ovrd=off  block_type=constant
      settings: block_version=11.4
  Constant4 : xbsIndex_r4/Constant  const=0  gui_display_data_type=Fixed-point  arith_type=Unsigned  n_bits=3  bin_pt=0  preci_type=Single  exp_width=8  frac_width=24  explicit_period=off  period=1  equ=P=C  opselect=C  inp2=PCIN>>17  opr=+  inp1=P  carry=CIN  dbl_ovrd=off  block_type=constant
      settings: block_version=11.4
  Constant5 : xbsIndex_r4/Constant  const=0  gui_display_data_type=Fixed-point  arith_type=Unsigned  n_bits=1  bin_pt=0  preci_type=Single  exp_width=8  frac_width=24  explicit_period=off  period=1  equ=P=C  opselect=C  inp2=PCIN>>17  opr=+  inp1=P  carry=CIN  dbl_ovrd=off  block_type=constant
      settings: block_version=11.4
  Constant6 : xbsIndex_r4/Constant  const=5  gui_display_data_type=Fixed-point  arith_type=Unsigned  n_bits=7  bin_pt=0  preci_type=Single  exp_width=8  frac_width=24  explicit_period=off  period=1  equ=P=C  opselect=C  inp2=PCIN>>17  opr=+  inp1=P  carry=CIN  dbl_ovrd=off  block_type=constant
      settings: block_version=11.4
  Constant7 : xbsIndex_r4/Constant  const=0  gui_display_data_type=Fixed-point  arith_type=Unsigned  n_bits=3  bin_pt=0  preci_type=Single  exp_width=8  frac_width=24  explicit_period=off  period=1  equ=P=C  opselect=C  inp2=PCIN>>17  opr=+  inp1=P  carry=CIN  dbl_ovrd=off  block_type=constant
      settings: block_version=11.4
  Constant8 : xbsIndex_r4/Constant  const=0  gui_display_data_type=Fixed-point  arith_type=Unsigned  n_bits=1  bin_pt=0  preci_type=Single  exp_width=8  frac_width=24  explicit_period=off  period=1  equ=P=C  opselect=C  inp2=PCIN>>17  opr=+  inp1=P  carry=CIN  dbl_ovrd=off  block_type=constant
      settings: block_version=11.4
  Convert : xbsIndex_r4/Convert  gui_display_data_type=Fixed-point  arith_type="Signed  (2's comp)"  n_bits=30  bin_pt=0  float_type=Single  exp_bits=8  fraction_bits=24  quantization=Truncate  overflow=Wrap  en=off  latency=0  dbl_ovrd=off  pipeline=off  block_type=convert
      settings: block_version=11.4
  Convert2 : xbsIndex_r4/Convert  gui_display_data_type=Fixed-point  arith_type="Signed  (2's comp)"  n_bits=30  bin_pt=0  float_type=Single  exp_bits=8  fraction_bits=24  quantization=Truncate  overflow=Wrap  en=off  latency=0  dbl_ovrd=off  pipeline=off  block_type=convert
      settings: block_version=11.4
  Convert3 : xbsIndex_r4/Convert  gui_display_data_type=Fixed-point  arith_type="Signed  (2's comp)"  n_bits=18  bin_pt=0  float_type=Single  exp_bits=8  fraction_bits=24  quantization=Truncate  overflow=Wrap  en=off  latency=0  dbl_ovrd=off  pipeline=off  block_type=convert
      settings: block_version=11.4
  Convert4 : xbsIndex_r4/Convert  gui_display_data_type=Fixed-point  arith_type="Signed  (2's comp)"  n_bits=18  bin_pt=0  float_type=Single  exp_bits=8  fraction_bits=24  quantization=Truncate  overflow=Wrap  en=off  latency=0  dbl_ovrd=off  pipeline=off  block_type=convert
      settings: block_version=11.4
  DSP48E_0 : xbsIndex_r4/DSP48E  use_a=Direct from A Port  use_b=Direct from B Port  reset_preg=off  pattern_from_creg=off  pattern='000000000000'  mask_from_creg=off  pattern_mask='3FFFFFFFFFFF'  sel_rounding_mask=Select mask  use_op=off  use_creg=off  rst_all=off  en_all=off  use_pcin=off  use_carrycascin=off  use_multsignin=off  use_carryout=off  use_patterndetect=off  use_patternbdetect=off  use_overflow=off  use_underflow=off  use_acout=off  use_bcout=off  use_pcout=on  use_multsignout=off  use_carrycascout=off  pipeline_a=1  pipeline_b=1  pipeline_acout=1  pipeline_bcout=1  pipeline_c=on  pipeline_p=on  pipeline_mult=on  pipeline_opmode=on  pipeline_alumode=on  pipeline_carryin=on  pipeline_carryinsel=on  rst_a=off  rst_b=off  rst_c=off  rst_mult=off  rst_p=off  rst_carry_in=off  rst_alumode=off  rst_ctrl=off  en_a1=off  en_a2=off  en_b1=off  en_b2=off  en_c=off  en_mult=off  en_p=off  en_carry_in=off  en_alumode=off  en_multcarryin=off  en_ctrl=off  use_synth_model=off  addsub_mode=ONE48  xl_useadderonly=off  block_type=dsp48e
      settings: block_version=11.4
  DSP48E_1 : xbsIndex_r4/DSP48E  use_a=Direct from A Port  use_b=Direct from B Port  reset_preg=off  pattern_from_creg=off  pattern='000000000000'  mask_from_creg=off  pattern_mask='3FFFFFFFFFFF'  sel_rounding_mask=Select mask  use_op=off  use_creg=off  rst_all=off  en_all=off  use_pcin=on  use_carrycascin=off  use_multsignin=off  use_carryout=off  use_patterndetect=off  use_patternbdetect=off  use_overflow=off  use_underflow=off  use_acout=off  use_bcout=off  use_pcout=off  use_multsignout=off  use_carrycascout=off  pipeline_a=2  pipeline_b=2  pipeline_acout=1  pipeline_bcout=1  pipeline_c=on  pipeline_p=on  pipeline_mult=on  pipeline_opmode=on  pipeline_alumode=on  pipeline_carryin=on  pipeline_carryinsel=on  rst_a=off  rst_b=off  rst_c=off  rst_mult=off  rst_p=off  rst_carry_in=off  rst_alumode=off  rst_ctrl=off  en_a1=off  en_a2=off  en_b1=off  en_b2=off  en_c=off  en_mult=off  en_p=off  en_carry_in=off  en_alumode=off  en_multcarryin=off  en_ctrl=off  use_synth_model=off  addsub_mode=ONE48  xl_useadderonly=off  block_type=dsp48e
      settings: block_version=11.4
  reinterp_imag : xbsIndex_r4/Reinterpret  force_arith_type=on  arith_type="Signed  (2's comp)"  force_bin_pt=off  bin_pt=0  block_type=reinterpret
      settings: infoedit="Changes signal type without altering the binary representation.   You can changed the signal between signed and unsigned, and relocate the binary point.<br><br>Hardware notes: In hardware this block costs nothing.<br><br>Example:  Suppose the input is 6 bits wide, signed, with 2 fractional bits, and the output is forced to unsigned with 0 fractional bits.  Then an input of -2.0 (1110.00 in binary 2's complement) becomes an output of 56 (111000 in binary)."
  reinterp_power : xbsIndex_r4/Reinterpret  force_arith_type=on  arith_type=Unsigned  force_bin_pt=on  bin_pt=34  block_type=reinterpret
      settings: infoedit="Changes signal type without altering the binary representation.   You can changed the signal between signed and unsigned, and relocate the binary point.<br><br>Hardware notes: In hardware this block costs nothing.<br><br>Example:  Suppose the input is 6 bits wide, signed, with 2 fractional bits, and the output is forced to unsigned with 0 fractional bits.  Then an input of -2.0 (1110.00 in binary 2's complement) becomes an output of 56 (111000 in binary)."
  reinterp_real : xbsIndex_r4/Reinterpret  force_arith_type=on  arith_type="Signed  (2's comp)"  force_bin_pt=off  bin_pt=0  block_type=reinterpret
      settings: infoedit="Changes signal type without altering the binary representation.   You can changed the signal between signed and unsigned, and relocate the binary point.<br><br>Hardware notes: In hardware this block costs nothing.<br><br>Example:  Suppose the input is 6 bits wide, signed, with 2 fractional bits, and the output is forced to unsigned with 0 fractional bits.  Then an input of -2.0 (1110.00 in binary 2's complement) becomes an output of 56 (111000 in binary)."
  slice_imag : xbsIndex_r4/Slice  nbits=18  boolean_output=off  mode=Lower Bit Location + Width  bit1=0  base1=MSB of Input  bit0=0  base0=LSB of Input  dbl_ovrd=off  block_type=slice
  slice_power : xbsIndex_r4/Slice  nbits=36  boolean_output=off  mode=Lower Bit Location + Width  bit1=0  base1=MSB of Input  bit0=0  base0=LSB of Input  dbl_ovrd=off  block_type=slice
  slice_real : xbsIndex_r4/Slice  nbits=18  boolean_output=off  mode=Upper Bit Location + Width  bit1=0  base1=MSB of Input  bit0=0  base0=LSB of Input  dbl_ovrd=off  block_type=slice
  p : Outport
  wires:
  reinterp_imag/1 -> Convert4/1, Convert2/1
  reinterp_real/1 -> Convert3/1, Convert/1
  c/1 -> slice_real/1, slice_imag/1
  slice_real/1 -> reinterp_real/1
  slice_power/1 -> reinterp_power/1
  DSP48E_1/1 -> slice_power/1
  slice_imag/1 -> reinterp_imag/1
  reinterp_power/1 -> p/1
  Constant4/1 -> DSP48E_1/7
  Constant5/1 -> DSP48E_1/6
  Constant2/1 -> DSP48E_1/5
  Constant3/1 -> DSP48E_1/4
  DSP48E_0/2 -> DSP48E_1/3
  Convert3/1 -> DSP48E_1/2
  Convert/1 -> DSP48E_1/1
  Constant7/1 -> DSP48E_0/6
  Constant8/1 -> DSP48E_0/5
  Constant1/1 -> DSP48E_0/4
  Constant6/1 -> DSP48E_0/3
  Convert4/1 -> DSP48E_0/2
  Convert2/1 -> DSP48E_0/1

== system casper_library_misc/triggered_counter/edge_detect ==
  in : Inport
  Delay : xbsIndex_r4/Delay  rst=off  infoeditControl=Selection of Reset will increase slice count due to use of real FFs and instead of SRLs  en=off  latency=1  dbl_ovrd=off  reg_retiming=on  block_type=delay
      settings: xl_area=[0, 0, 0, 0, 0, 0, 0]
  Inverter : xbsIndex_r4/Inverter  en=off  latency=0  dbl_ovrd=off  block_type=inv
      settings: xl_area=[0, 0, 0, 0, 0, 0, 0]
  edge_op : xbsIndex_r4/Logical  logical_function=NOR  inputs=2  en=off  latency=0  precision=Full  arith_type=Unsigned  n_bits=8  bin_pt=2  align_bp=on  dbl_ovrd=off  block_type=logical
      settings: xl_area=[0, 0, 0, 0, 0, 0, 0]
  out : Outport
  wires:
  Inverter/1 -> edge_op/1
  edge_op/1 -> out/1
  in/1 -> Inverter/1, Delay/1
  Delay/1 -> edge_op/2
